simulink subsystem "MotorDriveUnit_SystemThermal_refsub"  (R2025a)
settings: Solver=VariableStepAuto  StartTime=0.0  StopTime=10.0  RelTol=1e-3
undefined symbols (not defined in the file or in its folder): initial, Minus, motorDriveUnit, Plus
libraries: fl_lib x16, nesl_utility x10, ee_lib x1, sdl_lib x1
settings Model: Creator=isaacito  LastModifiedBy=isaacito
settings SolverCC: AlgebraicLoopSolver=TrustRegion
settings OptimizationCC: ReuseModelBlockBuffer=off
settings DebuggingCC: UnconnectedInputMsg=warning  UnconnectedOutputMsg=warning  UnconnectedLineMsg=warning
settings ModelReferenceCC: EnableRefExpFcnMdlSchedulingChecks=on
settings RTWCC: GPUComputeCapability=3.5  DLArmComputeVersion=19.05

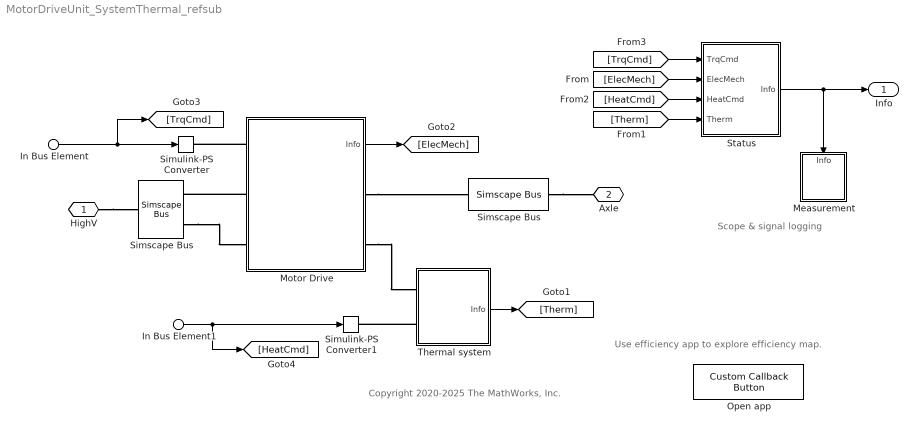
== system MotorDriveUnit_SystemThermal_refsub ==
  note: Copyright 2020-2025 The MathWorks, Inc.
  note: Scope & signal logging
  note: Use efficiency app to explore efficiency map.
  In Bus Element : Inport  PortName=Ctrl  Element=TrqCmd
      settings: AttributesFormatString=%<Unit>
  In Bus Element1 : Inport  PortName=Ctrl  Element=HeatCmd
      settings: AttributesFormatString=%<Unit>
  " Simscape Bus" : SimscapeBus  HierarchyStrings=Plus;Minus  ConnectionType=Bus: Bus_HighVoltage
      settings: AttributesFormatString=%<ConnectionType>
  Measurement : Subsystem
  Motor Drive : Subsystem
  Open app : CustomCallbackButton  Configuration="{\"components\":[{\"name\":\"BackgroundImageComponent\",\"settings\":{\"image\":{\"size\":[0,0],\"src\":\"default\",\"srcOrientation\":\"Right\"},\"position\":[0,0,1,1]}},{\"name\":\"ButtonStateComponent\",\"settings\":{\"buttonType\":\"momentary\",\"clickFcn\":\"MotorDriveUnitEfficiencyApp_SystemThermal\",\"onValue\":1,\"position\":[0,0,1,1],\"pressDelay\":\"500\",\"pressFcn\":\"\",\"repeatInterval\":\"0\",\"states\":[{\"horizontalAlignment\":\"center\",\"image\":{\"position\":[0,0,1,1],\"size\":[1,1],\"src\":\"default\",\"srcOrientation\":\"Right\"},\"label\":{\"color\":[0.01176470588,0.01176470588,0.01176470588,1],\"icon\":{\"size\":[0,0],\"src\":\"default\",\"srcOrientation\":\"Right\"},\"iconOffset\":0,\"iconPlacement\":\"left\",\"opacity\":1,\"show\":true,\"text\":{\"content\":\"Open app\",\"font\":\"Helvetica\"}},\"labelOffset\":[0,0],\"verticalAlignment\":\"middle\"},{\"horizontalAlignment\":\"center\",\"image\":{\"position\":[0,0,1,1],\"size\":[1,1],\"src\":\"default\",\"srcOrientation\":\"Right\"},\"label\":{\"color\":[0.01176470588,0.01176470588,0.01176470588,1],\"icon\":{\"size\":[0,0],\"src\":\"default\",\"srcOrientation\":\"Right\"},\"iconOffset\":0,\"iconPlacement\":\"left\",\"opacity\":1,\"show\":true,\"text\":{\"content\":\"Open app\",\"font\":\"Helvetica\"}},\"labelOffset\":[0,0],\"verticalAlignment\":\"middle\"},{\"horizontalAlignment\":\"center\",\"image\":{\"position\":[0,0,1,1],\"size\":[1,1],\"src\":\"default\",\"srcOrientation\":\"Right\"},\"label\":{\"color\":[0.01176470588,0.01176470588,0.01176470588,1],\"icon\":{\"size\":[0,0],\"src\":\"default\",\"srcOrientation\":\"Right\"},\"iconOffset\":0,\"iconPlacement\":\"left\",\"opacity\":1,\"show\":true,\"text\":{\"content\":\"Open app\",\"font\":\"Helvetica\"}},\"labelOffset\":[0,0],\"verticalAlignment\":\"middle\"},{\"horizontalAlignment\":\"center\",\"image\":{\"position\":[0,0,1,1],\"size\":[1,1],\"src\":\"default\",\"srcOrientation\":\"Right\"},\"label\":{\"color\":[0.01176470588,0.01176470588,0.01176470588,1],\"icon\":{\"size\":[0,0],\"src\":\"default\",\"srcOrientation\":\"Right\"},\"iconOffset\":0,\"iconPlacement\":\"left\",\"opacity\":1,\"show\":true,\"text\":{\"content\":\"Open app\",\"font\":\"Helvetica\"}},\"labelOffset\":[0,0],\"verticalAlignment\":\"middle\"}]}},{\"name\":\"ForegroundImageComponent\",\"settings\":{\"image\":{\"size\":[0,0],\"src\":\"default\",\"srcOrientation\":\"Right\"},\"isForeground\":1,\"position\":[0,0,1,1]}}],\"derived\":{\"blockParameters\":{\"AutoActivate\":true,\"ButtonText\":\"Open app\",\"ButtonType\":\"Momentary\",\"ClickFcn\":\"MotorDriveUnitEfficiencyApp_SystemThermal\",\"OnValue\":1,\"PressDelay\":\"500\",\"PressFcn\":\"\",\"RepeatInterval\":\"0\",\"fixedAspectRatio\":\"off\"}},\"settings\":{\"BindingType\":\"standalone\",\"autoActivate\":true,\"backgroundColor\":[244,244,244,1],\"backgroundOffset\":0.2,\"backgroundOpacity\":1,\"fixedAspectRatio\":\"off\",\"foregroundColor\":[0.01176470588,0.01176470588,0.01176470588,1],\"migratedFromLegacy\":true,\"useBackgroundColor\":true,\"variant\":\"callback\",\"version\":\"R2025a\"},\"type\":\"Button\"}"  CustomBackgroundColor="{\"color\":[0.9568627450980393,0.9568627450980393,0.9568627450980393],\"show\":true}"
  Simscape Bus : SimscapeBus  HierarchyStrings=AngSpd  ConnectionType=Bus: Bus_Rotational
      settings: AttributesFormatString=%<ConnectionType>
  Simulink-PS Converter : nesl_utility/Simulink-PS Converter  PhysicalDomain=network_engine_domain  SubClassName=ps_input  LeftPortType=input  RightPortType=output  PseudoPeriodic=off  Frequencies=[]  NoiseDistribution=none  NoiseParameters=[]  Unit=N*m  AffineConversion=off  FilteringAndDerivatives=filter  SimscapeFilterOrder=1  InputFilterTimeConstant=.001  UdotUserProvided=1
  Simulink-PS Converter1 : nesl_utility/Simulink-PS Converter  PhysicalDomain=network_engine_domain  SubClassName=ps_input  LeftPortType=input  RightPortType=output  PseudoPeriodic=off  Frequencies=[]  NoiseDistribution=none  NoiseParameters=[]  Unit=W  AffineConversion=off  FilteringAndDerivatives=provide  SimscapeFilterOrder=1  InputFilterTimeConstant=0.001  UdotUserProvided=0
  Status : Subsystem
  Thermal system : Subsystem
  HighV : PMIOPort  Side=Left
  Axle : PMIOPort  Port=2  Side=Right
  Info : Outport
  wires:
  In Bus Element/1 -> [TrqCmd], Simulink-PS Converter/1
  Status/1(Info) -> Measurement/1(Info), Info/1
  Motor Drive/1(Info) -> [ElecMech]
  In Bus Element1/1 -> [HeatCmd], Simulink-PS Converter1/1
  Thermal system/1(Info) -> [Therm]
  [Therm] -> Status/4(Therm)
  [HeatCmd] -> Status/3(HeatCmd)
  [TrqCmd] -> Status/1(TrqCmd)
  [ElecMech] -> Status/2(ElecMech)
  connections:
  HighV/RConn1 -- " Simscape Bus"/RConn1
  Simscape Bus/RConn1 -- Axle/RConn1
  Motor Drive/LConn2 -- " Simscape Bus"/LConn1
  Motor Drive/LConn1 -- Simulink-PS Converter/RConn1
  Motor Drive/RConn1 -- Simscape Bus/LConn1
  " Simscape Bus"/LConn2 -- Motor Drive/LConn3
  Thermal system/LConn2 -- Simulink-PS Converter1/RConn1
  Motor Drive/RConn2 -- Thermal system/LConn1

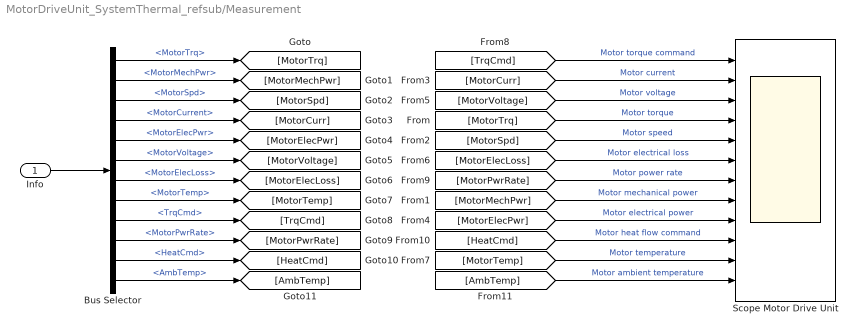
== system MotorDriveUnit_SystemThermal_refsub/Measurement ==
  Info : Inport
  Bus Selector : BusSelector  OutputSignals=MotorTrq,MotorMechPwr,MotorSpd,MotorCurrent,MotorElecPwr,MotorVoltage,MotorElecLoss,MotorTemp,TrqCmd,MotorPwrRate,HeatCmd,AmbTemp
  Scope Motor Drive Unit : Scope  NumInputPorts=12
  wires:
  Info/1 -> Bus Selector/1
  Bus Selector/1 -> [MotorTrq]  "<MotorTrq>"
  Bus Selector/2 -> [MotorMechPwr]  "<MotorMechPwr>"
  Bus Selector/3 -> [MotorSpd]  "<MotorSpd>"
  Bus Selector/4 -> [MotorCurr]  "<MotorCurrent>"
  Bus Selector/5 -> [MotorElecPwr]  "<MotorElecPwr>"
  Bus Selector/6 -> [MotorVoltage]  "<MotorVoltage>"
  Bus Selector/7 -> [MotorElecLoss]  "<MotorElecLoss>"
  Bus Selector/8 -> [MotorTemp]  "<MotorTemp>"
  Bus Selector/9 -> [TrqCmd]  "<TrqCmd>"
  Bus Selector/10 -> [MotorPwrRate]  "<MotorPwrRate>"
  Bus Selector/11 -> [HeatCmd]  "<HeatCmd>"
  Bus Selector/12 -> [AmbTemp]  "<AmbTemp>"
  [TrqCmd] -> Scope Motor Drive Unit/1  "Motor torque command"
  [MotorCurr] -> Scope Motor Drive Unit/2  "Motor current"
  [MotorVoltage] -> Scope Motor Drive Unit/3  "Motor voltage"
  [MotorTrq] -> Scope Motor Drive Unit/4  "Motor torque"
  [MotorSpd] -> Scope Motor Drive Unit/5  "Motor speed"
  [MotorElecLoss] -> Scope Motor Drive Unit/6  "Motor electrical loss"
  [MotorPwrRate] -> Scope Motor Drive Unit/7  "Motor power rate"
  [MotorMechPwr] -> Scope Motor Drive Unit/8  "Motor mechanical power"
  [MotorElecPwr] -> Scope Motor Drive Unit/9  "Motor electrical power"
  [HeatCmd] -> Scope Motor Drive Unit/10  "Motor heat flow command"
  [MotorTemp] -> Scope Motor Drive Unit/11  "Motor temperature"
  [AmbTemp] -> Scope Motor Drive Unit/12  "Motor ambient temperature"

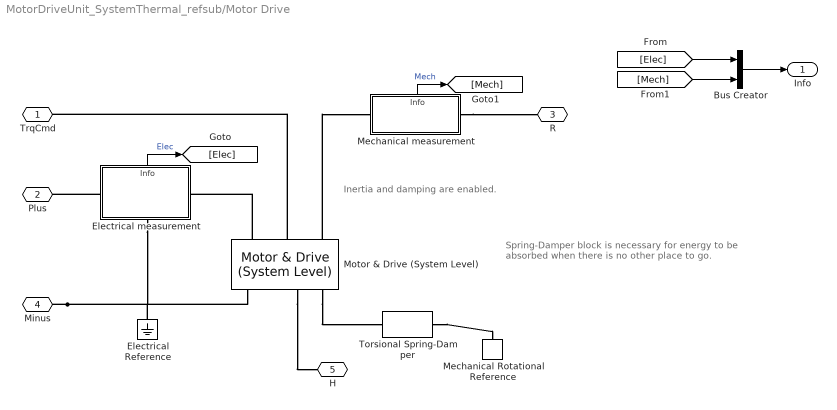
== system MotorDriveUnit_SystemThermal_refsub/Motor Drive ==
  note: Spring-Damper block is necessary
      | for energy to be absorbed when
      | there is no other place to go.
  note: Inertia and damping are enabled.
  Bus Creator : BusCreator  Inputs=2
  Electrical Reference : fl_lib/Electrical/Electrical Elements/Electrical Reference
  Electrical measurement : Subsystem
      settings: PortSchema="{\"entries\":[{\"content\":{\"sides\":[{\"content\":{\"connectorIds\":[\"LConn1\"]},\"type\":\"ConnectorPlacement.EquallySpacedRectSide\",\"uuid\":\"e7899a7c-736a-463f-af66-4f4d60778038\"},{\"content\":{\"connectorIds\":[\"RConn1\"],\"side\":\"RIGHT\"},\"type\":\"ConnectorPlacement.EquallySpacedRectSide\",\"uuid\":\"2a49f66b-d9e4-4ecc-9ee0-ab77c8229b93\"},{\"content\":{\"connectorIds\":[\"Out1\"],\"side\":\"TOP\"},\"type\":\"ConnectorPlacement.EquallySpacedRectSide\",\"uuid\":\"74dc25cc-80bc-4bc6-bed8-e6f8417263f8\"},{\"content\":{\"connectorIds\":[\"RConn2\"],\"side\":\"BOTTOM\"},\"type\":\"ConnectorPlacement.EquallySpacedRectSide\",\"uuid\":\"4e60d196-3559-4d10-956a-034c89d8b166\"}]},\"type\":\"ConnectorPlacement.EquallySpacedConnector\",\"uuid\":\"8c0a083e-e2f2-4f23-9344-a58537a7d46b\"}],\"packageUris\":[\"http://schema.mathworks.com/mf0/Connector/R2020b\"],\"version\":\"1.0\"}"
  Mechanical Rotational Reference : fl_lib/Mechanical/Rotational Elements/Mechanical Rotational Reference
  Mechanical measurement : Subsystem
      settings: PortSchema="{\"entries\":[{\"content\":{\"sides\":[{\"content\":{\"connectorIds\":[\"LConn1\"]},\"type\":\"ConnectorPlacement.EquallySpacedRectSide\",\"uuid\":\"5fa31342-f07e-4673-a9a7-985a7d429b77\"},{\"content\":{\"connectorIds\":[\"RConn1\"],\"side\":\"RIGHT\"},\"type\":\"ConnectorPlacement.EquallySpacedRectSide\",\"uuid\":\"9acd2d80-16ac-46ed-87fd-cbe927805b31\"},{\"content\":{\"connectorIds\":[\"Out1\"],\"side\":\"TOP\"},\"type\":\"ConnectorPlacement.EquallySpacedRectSide\",\"uuid\":\"4cbbe886-3c02-40e0-8c42-e8f0172dc845\"},{\"content\":{\"connectorIds\":[],\"side\":\"HIDDEN\"},\"type\":\"ConnectorPlacement.EquallySpacedRectSide\",\"uuid\":\"587bbe77-2244-497b-b5ee-9581dc02e6d6\"}]},\"type\":\"ConnectorPlacement.EquallySpacedConnector\",\"uuid\":\"7667f692-53dd-486a-a403-194e7923bdd7\"}],\"packageUris\":[\"http://schema.mathworks.com/mf0/Connector/R2020b\"],\"version\":\"1.0\"}"
  Motor & Drive (System Level) : ee_lib/Electromechanical/Motor & Drive (System Level)  torque_speed_param=ee.enum.electromech.envelope.torque_power  overtorque_param=ee.enum.electromech.overtorque.no  T_t=[.09, .08, .07, 0] N*m  T_t_intermittent=[.36, .32, .28, 0] N*m  T_t_2D=[.09, .09, .09; .08, .08, .08; .07, .07, .07; 0, 0, 0] N*m  T_t_intermittent_2D=[.36, .36, .36; .32, .32, .32; .28, .28, .28; 0, 0, 0] N*m  w_t=[0, 3750, 7500, 8000] rpm  vdc_t=[6, 12, 24] V  torque_max=motorDriveUnit.trqMax_Nm N*m  power_max=motorDriveUnit.powerMax_kW kW  torque_max_intermittent=0.4 N*m  power_max_intermittent=120 W  time_overtorque=30 s  time_recover=60 s  Tc=motorDriveUnit.responseTime_s s  EnableSwitch=simscape.enum.onoff.off  losses_param=1  eff=motorDriveUnit.efficiency_pct  w_eff=motorDriveUnit.spd_eff_rpm rpm  T_eff=motorDriveUnit.trq_eff_Nm N*m  Piron=motorDriveUnit.ironLoss_W W  Pbase=motorDriveUnit.fixedLoss_W W  w_eff_vec=motorDriveUnit.spdVec_rpm rpm  T_eff_vec=motorDriveUnit.trqVec_Nm N*m  v_eff_vec=[100, 250, 400] V  losses_mat=motorDriveUnit.electricalLosses_W W  efficiency_mat=[95, 95, 95, 95; 95, 95, 95, 95; 95, 95, 95, 95; 95, 95, 95, 95; 95, 95, 95, 95]  losses_mat_3D=ones(5, 4, 3) W  efficiency_mat_3D=95 * ones(5, 4, 3)  Res=0 Ohm  J=motorDriveUnit.rotorInertia_kg_m2 kg*m^2  lam=motorDriveUnit.rotorDamping_Nm_per_radps N*m/(rad/s)  speed0=initial.motorDriveUnit_RotorSpd_rpm rpm  faulted_specify=off  faulted_priority=None  faulted=0  faulted_nominal_specify=off  faulted_nominal_value=1  faulted_nominal_unit=1  isSwitchedOff_specify=off  isSwitchedOff_priority=None  isSwitchedOff=0  isSwitchedOff_nominal_specify=off  isSwitchedOff_nominal_value=1  isSwitchedOff_nominal_unit=1  torqueLimitContinuous_specify=off  torqueLimitContinuous_priority=None  torqueLimitContinuous=0 N*m  torqueLimitContinuous_nominal_specify=off  torqueLimitContinuous_nominal_value=1  torqueLimitContinuous_nominal_unit=N*m  alpha=3.93e-3 1/K  Tmeas=25 degC  Tmeas2=125 degC  losses_mat_T2=[1.49, 1.74, 2.49, 3.74; .42, .67, 1.42, 2.67; .06, .31, 1.06, 2.31; .42, .67, 1.42, 2.67; 1.49, 1.74, 2.49, 3.74] W  efficiency_mat_T2=[95, 95, 95, 95; 95, 95, 95, 95; 95, 95, 95, 95; 95, 95, 95, 95; 95, 95, 95, 95]  losses_mat_3D_T2=ones(5, 4, 3) W  efficiency_mat_3D_T2=95 * ones(5, 4, 3)  thermal_mass=motorDriveUnit.ThermalMass_J_per_K J/K  initial_temperature=initial.motorDriveUnit_Temperature_K degC
      settings: LogSimulationData=on  InternalSimscapePortConfiguration="{\"Bottom\":[],\"Left\":[{\"id\":\"Vp\",\"label\":\"+\",\"type\":\"foundation.electrical.electrical\"},{\"id\":\"Tr\",\"label\":\"Tr\",\"type\":\"input\"},{\"id\":\"R\",\"label\":\"R\",\"type\":\"foundation.mechanical.rotational.rotational\"}],\"Right\":[{\"id\":\"Vm\",\"label\":\"-\",\"type\":\"foundation.electrical.electrical\"},{\"id\":\"Omega\",\"label\":\"w\",\"type\":\"output\"},{\"id\":\"H\",\"label\":\"H\",\"type\":\"foundation.thermal.thermal\"},{\"id\":\"C\",\"label\":\"C\",\"type\":\"foundation.mechanical.rotational.rotational\"}],\"Top\":[]}"
  Torsional Spring-Damper : sdl_lib/Couplings & Drives/Torsional Spring-Damper  k=1000 N*m/rad  mu_visc=10000 m*N/rpm  trq_coulomb=0 N*m  static_kinetic_ratio=1.1  w_tol=0.1 rpm  model_hardstop=0  upper_bound=10 deg  lower_bound=-10 deg  hardstop_model=1  k_endstop=1e6 N*m/rad  D_endstop=10 N*m/(rad/s)  transition=0.001 rad  coeff_rest=0.7  w_tol_hardstop=0.1 rad/s  trq_tol=0.001 N*m  x0=0 deg
      settings: InternalSimscapePortConfiguration="{\"Bottom\":[],\"Left\":[{\"id\":\"R\",\"label\":\"R\",\"type\":\"foundation.mechanical.rotational.rotational\"}],\"Right\":[{\"id\":\"C\",\"label\":\"C\",\"type\":\"foundation.mechanical.rotational.rotational\"}],\"Top\":[]}"
  TrqCmd : PMIOPort  Side=Left
  Plus : PMIOPort  Port=2  Side=Left
  R : PMIOPort  Port=3  Side=Right
  Minus : PMIOPort  Port=4  Side=Left
  H : PMIOPort  Port=5  Side=Right
  Info : Outport
  wires:
  Bus Creator/1 -> Info/1
  [Mech] -> Bus Creator/2
  [Elec] -> Bus Creator/1
  Mechanical measurement/1(Info) -> [Mech]  "Mech"
  Electrical measurement/1(Info) -> [Elec]  "Elec"
  connections:
  Torsional Spring-Damper/RConn1 -- Mechanical Rotational Reference/LConn1
  Minus/RConn1 -- Motor & Drive (System Level)/RConn1 -- Electrical Reference/LConn1 -- Electrical measurement/RConn2
  Mechanical measurement/RConn1 -- R/RConn1
  Motor & Drive (System Level)/LConn1 -- Electrical measurement/RConn1
  Electrical measurement/LConn1 -- Plus/RConn1
  Motor & Drive (System Level)/LConn2 -- TrqCmd/RConn1
  Motor & Drive (System Level)/RConn4 -- Torsional Spring-Damper/LConn1
  Motor & Drive (System Level)/RConn3 -- H/RConn1
  Motor & Drive (System Level)/LConn3 -- Mechanical measurement/LConn1

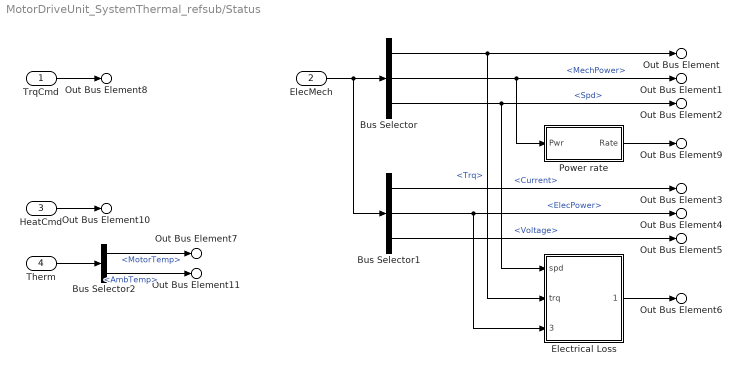
== system MotorDriveUnit_SystemThermal_refsub/Status ==
  TrqCmd : Inport
  ElecMech : Inport  Port=2
  HeatCmd : Inport  Port=3
  Therm : Inport  Port=4
  Bus Selector : BusSelector  OutputSignals=Mech.Trq,Mech.MechPower,Mech.Spd
  Bus Selector1 : BusSelector  OutputSignals=Elec.Current,Elec.ElecPower,Elec.Voltage
  Bus Selector2 : BusSelector  OutputSignals=MotorTemp,AmbTemp
  Electrical Loss : Subsystem
  Power rate : Subsystem
  Out Bus Element : Outport  PortName=Info  Element=MotorTrq
  Out Bus Element1 : Outport  PortName=Info  Element=MotorMechPwr
  Out Bus Element2 : Outport  PortName=Info  Element=MotorSpd
  Out Bus Element3 : Outport  PortName=Info  Element=MotorCurrent
  Out Bus Element4 : Outport  PortName=Info  Element=MotorElecPwr
  Out Bus Element5 : Outport  PortName=Info  Element=MotorVoltage
  Out Bus Element6 : Outport  PortName=Info  Element=MotorElecLoss
  Out Bus Element7 : Outport  PortName=Info  Element=MotorTemp
  Out Bus Element8 : Outport  PortName=Info  Element=TrqCmd
  Out Bus Element9 : Outport  PortName=Info  Element=MotorPwrRate
  Out Bus Element10 : Outport  PortName=Info  Element=HeatCmd
  Out Bus Element11 : Outport  PortName=Info  Element=AmbTemp
  wires:
  Power rate/1(Rate) -> Out Bus Element9/1
  Electrical Loss/1(elec_loss) -> Out Bus Element6/1
  Bus Selector1/3 -> Out Bus Element5/1  "<Voltage>"
  Bus Selector1/2 -> Electrical Loss/3(elec_pwr), Out Bus Element4/1  "<ElecPower>"
  Bus Selector1/1 -> Out Bus Element3/1  "<Current>"
  Bus Selector/3 -> Out Bus Element2/1, Electrical Loss/1(spd)  "<Spd>"
  Bus Selector/2 -> Out Bus Element1/1, Power rate/1(Pwr)  "<MechPower>"
  Bus Selector/1 -> Out Bus Element/1, Electrical Loss/2(trq)  "<Trq>"
  ElecMech/1 -> Bus Selector/1, Bus Selector1/1
  TrqCmd/1 -> Out Bus Element8/1
  HeatCmd/1 -> Out Bus Element10/1
  Therm/1 -> Bus Selector2/1
  Bus Selector2/1 -> Out Bus Element7/1  "<MotorTemp>"
  Bus Selector2/2 -> Out Bus Element11/1  "<AmbTemp>"

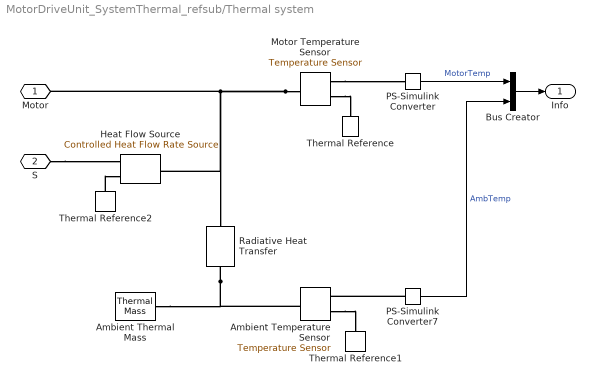
== system MotorDriveUnit_SystemThermal_refsub/Thermal system ==
  Ambient Temperature Sensor : fl_lib/Thermal/Thermal Sensors/Temperature Sensor  temperature_measure=foundation.enum.MeasurementReference.difference
  Ambient Thermal Mass : fl_lib/Thermal/Thermal Elements/Thermal Mass  mass_type=foundation.enum.constant_variable.constant  mass=motorDriveUnit.ambientMass_t t  sp_heat=motorDriveUnit.ambientSpecificHeat_J_per_Kkg J/(K*kg)  mass_min=1e-6 kg  num_ports=foundation.enum.numPorts2.one  m_specify=off  m_priority=High  m=1 kg  m_nominal_specify=off  m_nominal_value=1  m_nominal_unit=kg  T_specify=on  T_priority=High  T=initial.ambientTemp_K K  T_nominal_specify=off  T_nominal_value=1  T_nominal_unit=K  Q_specify=off  Q_priority=None  Q=0 W  Q_nominal_specify=off  Q_nominal_value=1  Q_nominal_unit=W
      settings: AttributesFormatString=|
      | Initial: %<T> [%<T_unit>]
      | Priority: %<T_priority>
  Bus Creator : BusCreator  Inputs=2
  Heat Flow Source : fl_lib/Thermal/Thermal Sources/Controlled Heat Flow Rate Source
  Motor Temperature Sensor : fl_lib/Thermal/Thermal Sensors/Temperature Sensor  temperature_measure=foundation.enum.MeasurementReference.difference
  PS-Simulink Converter : nesl_utility/PS-Simulink Converter  PhysicalDomain=network_engine_domain  SubClassName=ps_output  LeftPortType=input  RightPortType=output  PseudoPeriodic=off  Frequencies=[]  VectorFormat=inherit  Unit=degC  AffineConversion=on
  PS-Simulink Converter7 : nesl_utility/PS-Simulink Converter  PhysicalDomain=network_engine_domain  SubClassName=ps_output  LeftPortType=input  RightPortType=output  PseudoPeriodic=off  Frequencies=[]  VectorFormat=inherit  Unit=degC  AffineConversion=on
  Radiative Heat Transfer : fl_lib/Thermal/Thermal Elements/Radiative Heat Transfer  area=motorDriveUnit.RadiationArea_m2 m^2  rad_tr_coeff=motorDriveUnit.RadiationCoeff_W_per_K4m2 W/(K^4*m^2)  T_specify=off  T_priority=None  T=0 K  T_nominal_specify=off  T_nominal_value=1  T_nominal_unit=K  Q_specify=off  Q_priority=None  Q=0 W  Q_nominal_specify=off  Q_nominal_value=1  Q_nominal_unit=W
      settings: InternalSimscapePortConfiguration="{\"Bottom\":[],\"Left\":[{\"id\":\"A\",\"label\":\"A\",\"type\":\"foundation.thermal.thermal\"}],\"Right\":[{\"id\":\"B\",\"label\":\"B\",\"type\":\"foundation.thermal.thermal\"}],\"Top\":[]}"
  Thermal Reference : fl_lib/Thermal/Thermal Elements/Thermal Reference
  Thermal Reference1 : fl_lib/Thermal/Thermal Elements/Thermal Reference
  Thermal Reference2 : fl_lib/Thermal/Thermal Elements/Thermal Reference
  Motor : PMIOPort  Side=Left
  S : PMIOPort  Port=2  Side=Left
  Info : Outport
  wires:
  PS-Simulink Converter/1 -> Bus Creator/1  "MotorTemp"
  PS-Simulink Converter7/1 -> Bus Creator/2  "AmbTemp"
  Bus Creator/1 -> Info/1
  connections:
  Motor Temperature Sensor/RConn2 -- PS-Simulink Converter/LConn1
  Motor Temperature Sensor/LConn1 -- Motor/RConn1 -- Heat Flow Source/LConn1 -- Radiative Heat Transfer/RConn1
  Motor Temperature Sensor/RConn1 -- Thermal Reference/LConn1
  Radiative Heat Transfer/LConn1 -- Ambient Temperature Sensor/LConn1 -- Ambient Thermal Mass/LConn1
  Ambient Temperature Sensor/RConn1 -- Thermal Reference1/LConn1
  PS-Simulink Converter7/LConn1 -- Ambient Temperature Sensor/RConn2
  S/RConn1 -- Heat Flow Source/RConn1
  Thermal Reference2/LConn1 -- Heat Flow Source/RConn2

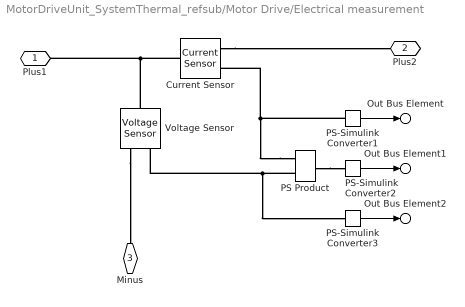
== system MotorDriveUnit_SystemThermal_refsub/Motor Drive/Electrical measurement ==
  Current Sensor : fl_lib/Electrical/Electrical Sensors/Current Sensor
  PS Product : fl_lib/Physical Signals/Functions/PS Product
  PS-Simulink Converter1 : nesl_utility/PS-Simulink Converter  PhysicalDomain=network_engine_domain  SubClassName=ps_output  LeftPortType=input  RightPortType=output  PseudoPeriodic=off  Frequencies=[]  VectorFormat=1-D array  Unit=A  AffineConversion=off
  PS-Simulink Converter2 : nesl_utility/PS-Simulink Converter  PhysicalDomain=network_engine_domain  SubClassName=ps_output  LeftPortType=input  RightPortType=output  PseudoPeriodic=off  Frequencies=[]  VectorFormat=1-D array  Unit=kW  AffineConversion=off
  PS-Simulink Converter3 : nesl_utility/PS-Simulink Converter  PhysicalDomain=network_engine_domain  SubClassName=ps_output  LeftPortType=input  RightPortType=output  PseudoPeriodic=off  Frequencies=[]  VectorFormat=1-D array  Unit=V  AffineConversion=off
  Voltage Sensor : fl_lib/Electrical/Electrical Sensors/Voltage Sensor
  Plus1 : PMIOPort  Side=Left
  Plus2 : PMIOPort  Port=2  Side=Right
  Minus : PMIOPort  Port=3  Side=Right
  Out Bus Element : Outport  PortName=Info  Element=Current
  Out Bus Element1 : Outport  PortName=Info  Element=ElecPower
  Out Bus Element2 : Outport  PortName=Info  Element=Voltage
  wires:
  PS-Simulink Converter1/1 -> Out Bus Element/1
  PS-Simulink Converter3/1 -> Out Bus Element2/1
  PS-Simulink Converter2/1 -> Out Bus Element1/1
  connections:
  PS Product/RConn1 -- PS-Simulink Converter2/LConn1
  PS Product/LConn1 -- Current Sensor/RConn1 -- PS-Simulink Converter1/LConn1
  Voltage Sensor/RConn1 -- PS-Simulink Converter3/LConn1 -- PS Product/LConn2
  Voltage Sensor/LConn1 -- Plus1/RConn1 -- Current Sensor/LConn1
  Current Sensor/RConn2 -- Plus2/RConn1
  Voltage Sensor/RConn2 -- Minus/RConn1

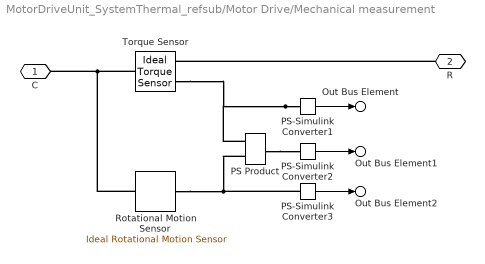
== system MotorDriveUnit_SystemThermal_refsub/Motor Drive/Mechanical measurement ==
  PS Product : fl_lib/Physical Signals/Functions/PS Product
  PS-Simulink Converter1 : nesl_utility/PS-Simulink Converter  PhysicalDomain=network_engine_domain  SubClassName=ps_output  LeftPortType=input  RightPortType=output  PseudoPeriodic=off  Frequencies=[]  VectorFormat=1-D array  Unit=N*m  AffineConversion=off
  PS-Simulink Converter2 : nesl_utility/PS-Simulink Converter  PhysicalDomain=network_engine_domain  SubClassName=ps_output  LeftPortType=input  RightPortType=output  PseudoPeriodic=off  Frequencies=[]  VectorFormat=1-D array  Unit=kW  AffineConversion=off
  PS-Simulink Converter3 : nesl_utility/PS-Simulink Converter  PhysicalDomain=network_engine_domain  SubClassName=ps_output  LeftPortType=input  RightPortType=output  PseudoPeriodic=off  Frequencies=[]  VectorFormat=1-D array  Unit=rpm  AffineConversion=off
  Rotational Motion Sensor : fl_lib/Mechanical/Mechanical Sensors/Ideal Rotational Motion Sensor  reference=foundation.enum.MeasurementReference.absolute  acceleration_port=false  velocity_port=true  position_port=false  wrap_angle=simscape.enum.onoff.off  offset=0 rad
      settings: InternalSimscapePortConfiguration="{\"Bottom\":[],\"Left\":[{\"id\":\"R\",\"label\":\"R\",\"type\":\"foundation.mechanical.rotational.rotational\"}],\"Right\":[{\"id\":\"W\",\"label\":\"W\",\"type\":\"output\"}],\"Top\":[]}"
  Torque Sensor : fl_lib/Mechanical/Mechanical Sensors/Ideal Torque Sensor
  C : PMIOPort  Side=Left
  R : PMIOPort  Port=2  Side=Right
  Out Bus Element : Outport  PortName=Info  Element=Trq
  Out Bus Element1 : Outport  PortName=Info  Element=MechPower
  Out Bus Element2 : Outport  PortName=Info  Element=Spd
  wires:
  PS-Simulink Converter1/1 -> Out Bus Element/1
  PS-Simulink Converter2/1 -> Out Bus Element1/1
  PS-Simulink Converter3/1 -> Out Bus Element2/1
  connections:
  PS Product/RConn1 -- PS-Simulink Converter2/LConn1
  PS-Simulink Converter3/LConn1 -- Rotational Motion Sensor/RConn1 -- PS Product/LConn2
  Torque Sensor/LConn1 -- Rotational Motion Sensor/LConn1 -- C/RConn1
  R/RConn1 -- Torque Sensor/RConn1
  PS-Simulink Converter1/LConn1 -- Torque Sensor/RConn2 -- PS Product/LConn1

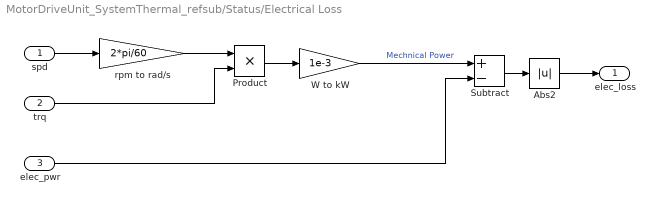
== system MotorDriveUnit_SystemThermal_refsub/Status/Electrical Loss ==
  spd : Inport  Unit=rpm
      settings: AttributesFormatString=%<Unit>
  trq : Inport  Port=2  Unit=N*m
      settings: AttributesFormatString=%<Unit>
  elec_pwr : Inport  Port=3  Unit=kW
      settings: AttributesFormatString=%<Unit>
  Abs2 : Abs  ZeroCross=off  SaturateOnIntegerOverflow=off
  Product : Product
  Subtract : Sum  Inputs=+-
  W to kW : Gain  Gain=1e-3
  rpm to rad/s : Gain  Gain=2*pi/60
  elec_loss : Outport  Unit=kW
      settings: AttributesFormatString=%<Unit>
  wires:
  W to kW/1 -> Subtract/1  "Mechnical Power"
  Abs2/1 -> elec_loss/1
  Subtract/1 -> Abs2/1
  elec_pwr/1 -> Subtract/2
  Product/1 -> W to kW/1
  rpm to rad/s/1 -> Product/1
  spd/1 -> rpm to rad/s/1
  trq/1 -> Product/2

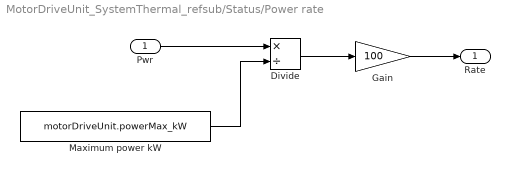
== system MotorDriveUnit_SystemThermal_refsub/Status/Power rate ==
  Pwr : Inport  Unit=kW
      settings: AttributesFormatString=%<Unit>
  Divide : Product  Inputs=*/
  Gain : Gain  Gain=100
  Maximum power kW : Constant  Value=motorDriveUnit.powerMax_kW
  Rate : Outport  Unit=%
  wires:
  Maximum power kW/1 -> Divide/2
  Gain/1 -> Rate/1
  Divide/1 -> Gain/1
  Pwr/1 -> Divide/1
